simulink model "Me492CasterM2"  (R2026b)
settings: Solver=ode4  StopTime=4  FixedStep=solver_step_s
model workspace (MAT data in the model file):
  caster_contact_enabled = 1
  command_sample_dt_s = 0.01
  initial_state = [-0.08; 0; 0; 0; 0; 0; 0; 0; 0; 0; 0; 0; 0]
  p_vector = [16; 0.6; 0.45; 0.0015; 0.0045; 0.00045; -0.08; 0; 0.12; 0.075; 0.38; 0.04; 0.05; -0.18; 0; 9.81; 0.6; 0.6; 300; 600; 200; 250; 0.008; 0.012; 0.00025; 0.0001; 0.004; 0.006; 0.1; 0.08; 0.002; 0.12]
  solver_step_s = 0.0005
  torque_array = [0 0.01 0.02 0.03 0.04 0.05 0.06 0.07 0.08 0.09 0.1 0.11 ... (1203 elements, 401x3)]
settings Model: Creator=lelfs  LastModifiedBy=lelfs
settings DataIOCC: SaveOutput=off  SignalLogging=off

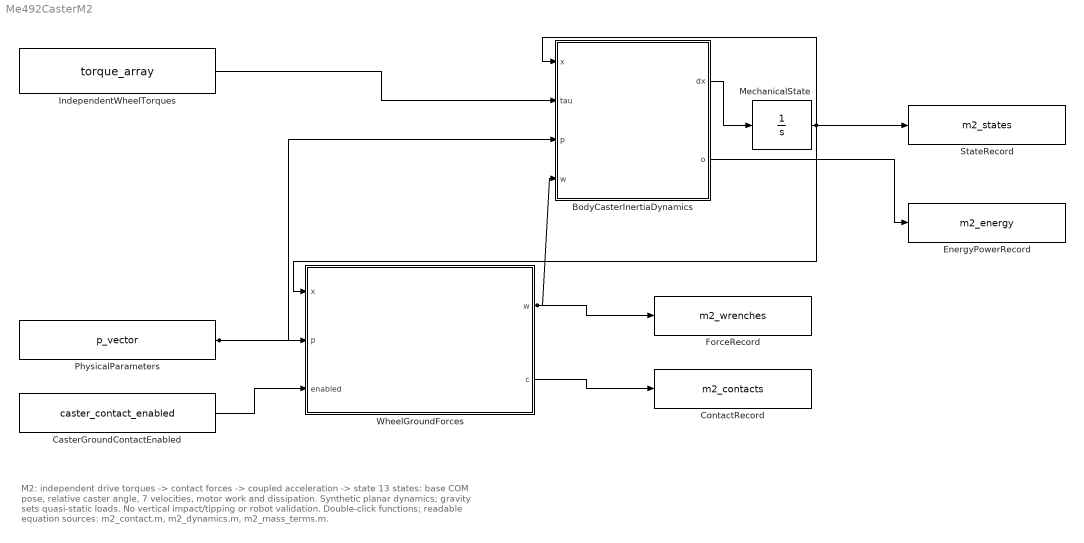
== system Me492CasterM2 ==
  note: M2: independent drive torques -> contact forces -> coupled acceleration -> state
      | 13 states: base COM pose, relative caster angle, 7 velocities, motor work and dissipation.
      | Synthetic planar dynamics; gravity sets quasi-static loads. No vertical impact/tipping or robot validation.
      | Double-click functions; readable equation sources: m2_contact.m, m2_dynamics.m, m2_mass_terms.m.
  BodyCasterInertiaDynamics : MATLAB Function  TreatAsAtomicUnit=on
  CasterGroundContactEnabled : Constant  Value=caster_contact_enabled
  ContactRecord : ToWorkspace  VariableName=m2_contacts  SaveFormat=Timeseries  SampleTime=-1
  EnergyPowerRecord : ToWorkspace  VariableName=m2_energy  SaveFormat=Timeseries  SampleTime=-1
  ForceRecord : ToWorkspace  VariableName=m2_wrenches  SaveFormat=Timeseries  SampleTime=-1
  IndependentWheelTorques : FromWorkspace  VariableName=torque_array  SampleTime=command_sample_dt_s  Interpolate=off  OutputAfterFinalValue=Holding final value
  MechanicalState : Integrator  InitialCondition=initial_state
  PhysicalParameters : Constant  Value=p_vector
  StateRecord : ToWorkspace  VariableName=m2_states  SaveFormat=Timeseries  SampleTime=-1
  WheelGroundForces : MATLAB Function  TreatAsAtomicUnit=on
  wires:
  MechanicalState/1 -> WheelGroundForces/1(x), BodyCasterInertiaDynamics/1(x), StateRecord/1
  PhysicalParameters/1 -> WheelGroundForces/2(p), BodyCasterInertiaDynamics/3(p)
  CasterGroundContactEnabled/1 -> WheelGroundForces/3(enabled)
  IndependentWheelTorques/1 -> BodyCasterInertiaDynamics/2(tau)
  WheelGroundForces/1(w) -> BodyCasterInertiaDynamics/4(w), ForceRecord/1
  BodyCasterInertiaDynamics/1(dx) -> MechanicalState/1
  WheelGroundForces/2(c) -> ContactRecord/1
  BodyCasterInertiaDynamics/2(o) -> EnergyPowerRecord/1

== matlab function Me492CasterM2/BodyCasterInertiaDynamics ==
  data: x input; dx output; tau input; p input; w input; o output
function [dx,o] = dynamics(x,tau,p,w)
%#codegen
[dx,o]=m2_dynamics(x,tau(:),p,w);
end

== matlab function Me492CasterM2/WheelGroundForces ==
  data: x input; w output; p input; enabled input; c output
function [w,c] = contact(x,p,enabled)
%#codegen
[w,c]=m2_contact(x,p,enabled);
end
